simulink model "I2Ctest"  (Simulink 7.1)
settings: Solver=FixedStepDiscrete  StartTime=0.0  StopTime=10.0  FixedStep=0.01  RelTol=1e-3
libraries: dsPICdrivers x4
CloseFcn:
  | rtwprivate ssgencode ModelCloseRequest ADC2PWM
settings Model: Creator=Lubin  LastModifiedBy=Gabe
settings OptimizationCC: OptimizeModelRefInitCode=on  LifeSpan=1
settings DebuggingCC: SaveWithParameterizedLinksMsg=none  SignalResolutionControl=TryResolveAllWithWarning
settings HardwareCC: ProdBitPerInt=16  ProdEndianess=LittleEndian  ProdWordSize=16  ProdHWDeviceType=16-bit Generic  TargetHWDeviceType=32-bit Generic
settings RTWCC: SystemTargetFile=dspic.tlc  TemplateMakefile=dspic_pic30_gcc.tmf  PostCodeGenCommand=dsPIC_Compile()  Description=Embedded Target for Microchip dsPIC (real-time)  ProcessScript=dspic_make_rtw_hook
settings CodeAppCC: IgnoreCustomStorageClasses=off
settings STFCustomTargetCC: ModelReferenceCompliant=off  IncludeMdlTerminateFcn=off  CombineOutputUpdateFcns=on  SuppressErrorStatus=on  ERTCustomFileBanners=on  SupportContinuousTime=off  SupportNonInlinedSFcns=off  SystemTargetFile=dspic.tlc
settings ERTTargetCC: ModelReferenceCompliant=off  CompOptLevelCompliant=off  IncludeMdlTerminateFcn=off  SuppressErrorStatus=on  ERTFirstTimeCompliant=off  ModelStepFunctionPrototypeControlCompliant=off  InlinedParameterPlacement=NonHierarchical  ERTSrcFileBannerTemplate=dsPIC_code_template.cgt  ERTHdrFileBannerTemplate=dsPIC_code_template.cgt  ERTDataSrcFileTemplate=dsPIC_code_template.cgt  ERTDataHdrFileTemplate=dsPIC_code_template.cgt  ERTCustomFileTemplate=dsPIC_main.tlc
settings CustomProperty: DataType=string  Value=C:\PROGRA~1\MATLAB\R2008a\bin\win32\gmake

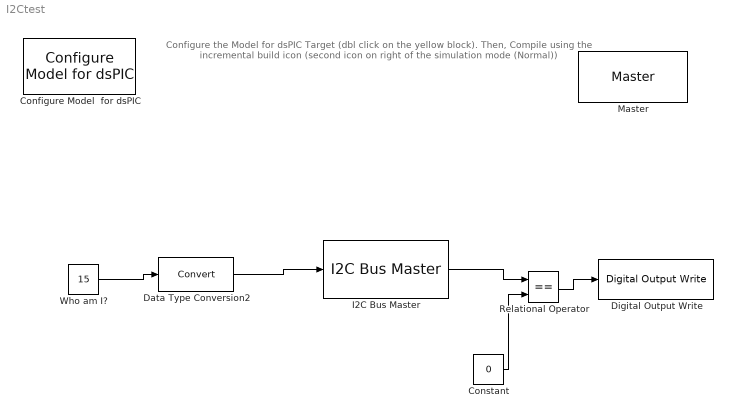
== system I2Ctest ==
  note: Configure the Model for dsPIC Target (dbl click on the yellow block).
      | Then, Compile using the incremental build icon
      | (second icon on right of the simulation mode (Normal))
  Configure Model  for dsPIC : dsPICdrivers/Simulink Configuration/Configure Model  for dsPIC
  Constant : Constant  Value=0  OutDataType=sfix(16)  OutScaling=2^0
  Data Type Conversion2 : DataTypeConversion  OutDataType=sfix(16)  OutScaling=2^0
  Digital Output Write : dsPICdrivers/Digital I//O/Digital Output Write  Tag=dsPIC_Digital_Output  Priority=5  PORT=B  Pin=[0]  Simultaneous=off  OrderingInOutPopup=None
  I2C Bus Master : dsPICdrivers/BUS I2C/I2C Bus Master  Tag=dsPIC_I2C_Master  NumI2C=1  Sequence='S A058 W Sr A059 Rnack P'  InitializeOnceOnly=When PIC is initialized (only once)  Enable=off  WaitAfterEnable=1  Disable=off  AdressNbrBits=7 bits  I2CBusFreq=227  SlewRate=off  SMBUSThreshold=off  OutputErrorFlag=off  SampleTime=-1  OrderingInOutPopup=None  Info=Fscl = 31.4108 KHz
  Master : dsPICdrivers/Master  Tag=dsPIC_MASTER  Priority=1  TimeStepType=Timer1  picType=30f3012  fcy=7.37e6  Quartz_33f=5e6  PLLActive_33f=off  fcyDesired_33f=0  tmr1="[8  9212  -0.0054274]"  tmr1Info="Time Step : 0.010001  ;   Error : -0.0054274%  PR1=9212"  tmr2345="[0  0]"  tmr2345cfg=[-1 -1]  IOautoConf=on  typePort="[ 0   0   0   0   0   0   0   0   0   0   0   0   0   0   0   0  10   0   0   0  20  20   0   0   0   0   0   0   0   0   0   0   0   0   0   0   0   0   0   0   0   0   0   0   0   0   0   0   0   0   0   0   0   0   0   0   0   0   0   0   0   0   0   0   0   0   0   0   0   0   0   0   0   0   0   0   0   0   0   0   0   0   0   0   0   0   0   0   0   0   0   0   0   0   0   0   0   0   0   0   0   0   0   0   0   0   0   0   0   0   0   0 ]"  TRIS="[ 65535  65534  65535  65535  65535  65535  65535 ]"  ADPCFG=1  MasterBusyPort=None  MasterOverloadPort=None  FOSC=FRC_PLL4  ClockSwitchMonitor=Both disabled  TempProtection_33f=TEMP_ON  FPBOR=PBOR_OFF  PWRT=PWRT_OFF  MCLR=MCLR_DIS  PowerSave=off  OverrideFcy=off  NewFcy=1e6
  Relational Operator : RelationalOperator  Operator===  LogicOutDataTypeMode=boolean  OutDataTypeStr=boolean
  Who am I? : Constant  Value=15  OutDataType=sfix(16)  OutScaling=2^0
  wires:
  Who am I?/1 -> Data Type Conversion2/1
  Data Type Conversion2/1 -> I2C Bus Master/1
  I2C Bus Master/1 -> Relational Operator/1
  Relational Operator/1 -> Digital Output Write/1
  Constant/1 -> Relational Operator/2
